simulink model "system_discrete"  (R2026b)
settings: Solver=VariableStepAuto  StopTime=50.0
values from neighbouring files (symbols this model uses):
  A_d = sys_d.A    [controller_observer_design.m]    (also in setup.m)
  B_d = sys_d.B    [controller_observer_design.m]    (also in setup.m)
  C_d = sys_d.C    [controller_observer_design.m]    (also in setup.m)
  K_discrete = dlqr(A_d,B_d,Q*Ts,R*Ts)    [controller_observer_design.m]    (also in setup.m)
  omega2u = [k, k, k, k; L*k, 0, -L*k, 0; 0, L*k, 0, -L*k; b, -b, b, -b]    [controller_observer_design.m]    (also in notes.m; setup.m)
  parameters =     [parameters.mat]
  Ts = 0.01    [controller_observer_design.m]    (also in setup.m)
  u2omega = (1/(4*b*L*k)) * [b*L, 2*b, 0, L*k; b*L, 0, 2*b, -L*k; b*L, -2*b, 0, L*k; b*L, 0, -2*b, -L*k]    [controller_observer_design.m]    (also in notes.m; setup.m)
undefined symbols (not defined in the file or in its folder): L_discrete
settings Model: Creator=elton  LastModifiedBy=elton

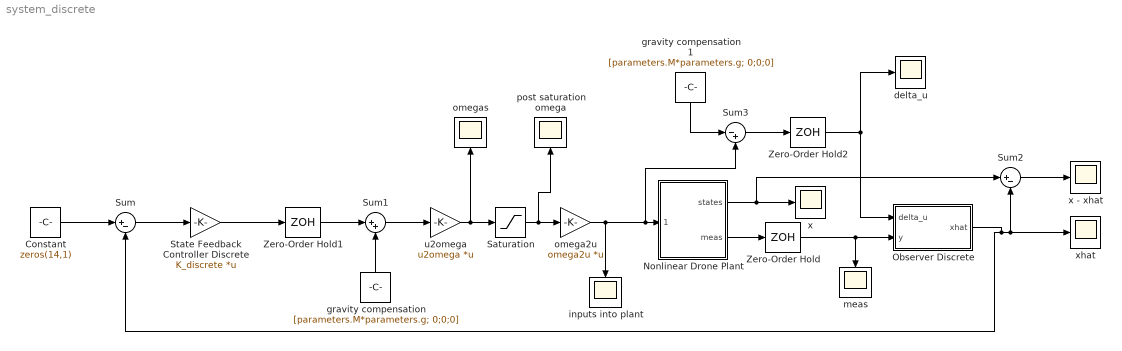
== system system_discrete ==
  Constant : Constant  Value=zeros(14,1)
  Nonlinear Drone Plant : Subsystem
  Observer Discrete : Subsystem
  Saturation : Saturate  UpperLimit=250000  LowerLimit=-250000
  State Feedback Controller Discrete : Gain  Gain=K_discrete  Multiplication=Matrix(K*u)
  Sum : Sum  Inputs=|+-
  Sum1 : Sum  Inputs=|++
  Sum2 : Sum  Inputs=|+-
  Sum3 : Sum  Inputs=|-+
  Zero-Order Hold : ZeroOrderHold  SampleTime=Ts
  Zero-Order Hold1 : ZeroOrderHold  SampleTime=Ts
  Zero-Order Hold2 : ZeroOrderHold  SampleTime=Ts
  delta_u : Scope
      settings: ActiveDisplayYMinimum=-0.1401923631580794  ActiveDisplayYMaximum=0.1652403175832419
  gravity compensation : Constant  Value=[parameters.M*parameters.g; 0;0;0]
  gravity compensation1 : Constant  Value=[parameters.M*parameters.g; 0;0;0]
  inputs into plant : Scope
      settings: ActiveDisplayYMinimum=-2.3883084159431922  ActiveDisplayYMaximum=20.39828479264926  DataLoggingVariableName=ScopeData7
  meas : Scope
      settings: ActiveDisplayYMinimum=-955.77756320006051  ActiveDisplayYMaximum=3490.5526217286788
  omega2u : Gain  Gain=omega2u  Multiplication=Matrix(K*u)
  omegas : Scope
      settings: ActiveDisplayYMinimum=134655.3751089205  ActiveDisplayYMaximum=149544.1079274721  DataLoggingVariableName=ScopeData8
  post saturation omega : Scope
      settings: ActiveDisplayYMinimum=131190.65308987262  ActiveDisplayYMaximum=153058.63070765982  DataLoggingVariableName=ScopeData9
  u2omega : Gain  Gain=u2omega  Multiplication=Matrix(K*u)
  x : Scope
      settings: ActiveDisplayYMinimum=-3.9919495753559691  ActiveDisplayYMaximum=4.13956426955115  DataLoggingVariableName=ScopeData6
  x - xhat : Scope
      settings: ActiveDisplayYMinimum=-0.067708761293840292  ActiveDisplayYMaximum=0.11746078567035534  DataLoggingVariableName=ScopeData2
  xhat : Scope
      settings: ActiveDisplayYMinimum=-0.014697140701710146  ActiveDisplayYMaximum=0.014411144567585507  DataLoggingVariableName=ScopeData3
  wires:
  Sum3/1 -> Zero-Order Hold2/1
  Sum1/1 -> u2omega/1
  State Feedback Controller Discrete/1 -> Zero-Order Hold1/1
  u2omega/1 -> Saturation/1, omegas/1
  omega2u/1 -> Sum3/2, Nonlinear Drone Plant/1(inputs), inputs into plant/1
  Observer Discrete/1(xhat) -> xhat/1, Sum2/2, Sum/2
  Nonlinear Drone Plant/1(states) -> x/1, Sum2/1
  Zero-Order Hold2/1 -> delta_u/1, Observer Discrete/1(delta_u)
  gravity compensation/1 -> Sum1/2
  Saturation/1 -> post saturation omega/1, omega2u/1
  gravity compensation1/1 -> Sum3/1
  Sum/1 -> State Feedback Controller Discrete/1
  Zero-Order Hold/1 -> meas/1, Observer Discrete/2(y)
  Sum2/1 -> x - xhat/1
  Zero-Order Hold1/1 -> Sum1/1
  Nonlinear Drone Plant/2(meas) -> Zero-Order Hold/1
  Constant/1 -> Sum/1

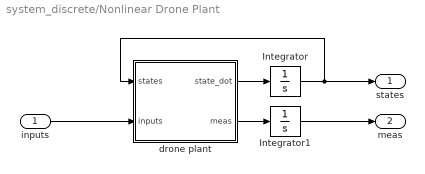
== system system_discrete/Nonlinear Drone Plant ==
  inputs : Inport
  Integrator : Integrator  InitialCondition=[zeros(12,1);0.049;0]
  Integrator1 : Integrator  InitialCondition=zeros(6,1)
  drone plant : MATLAB Function  TreatAsAtomicUnit=on
  states : Outport
  meas : Outport  Port=2
  wires:
  drone plant/1(state_dot) -> Integrator/1
  Integrator/1 -> states/1, drone plant/1(states)
  inputs/1 -> drone plant/2(inputs)
  Integrator1/1 -> meas/1
  drone plant/2(meas) -> Integrator1/1

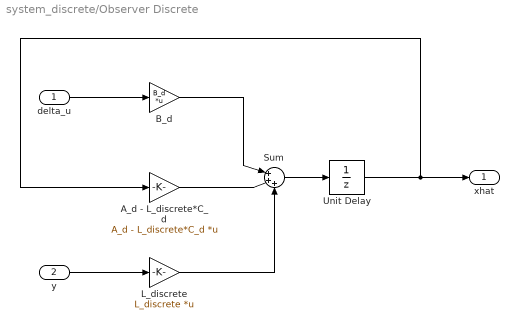
== system system_discrete/Observer Discrete ==
  delta_u : Inport
  y : Inport  Port=2
  A_d - L_discrete*C_d : Gain  Gain=A_d - L_discrete*C_d  Multiplication=Matrix(K*u)
  B_d : Gain  Gain=B_d  Multiplication=Matrix(K*u)
  L_discrete : Gain  Gain=L_discrete  Multiplication=Matrix(K*u)
  Sum : Sum  Inputs=|+++
  Unit Delay : UnitDelay  InitialCondition=zeros(14,1)  SampleTime=-1
  xhat : Outport
  wires:
  y/1 -> L_discrete/1
  B_d/1 -> Sum/1
  L_discrete/1 -> Sum/3
  A_d - L_discrete*C_d/1 -> Sum/2
  Sum/1 -> Unit Delay/1
  Unit Delay/1 -> A_d - L_discrete*C_d/1, xhat/1
  delta_u/1 -> B_d/1

== matlab function system_discrete/Nonlinear Drone Plant/drone plant ==
  data: states input size=14; inputs input size=4; state_dot output size=14; parameters parameter; meas output
%% non-linear state space
function [state_dot, meas]  = nonlin_state_space(states, inputs, parameters)
m     = parameters.m;
m_p    = parameters.m_p;
M     = m + m_p;
g     = parameters.g;
l     = parameters.l;
k_D    = parameters.k_D;
I_xx  = parameters.I_xx;
I_yy  = parameters.I_yy;
I_zz  = parameters.I_zz;

xi = states(1:3);
xi_dot = states(4:6);
eta = states(7:9);
nu = states(10:12);
alpha = states(13);
alpha_dot = states(14);

u_T = inputs(1);
tau = inputs(2:4);

x_dot = xi_dot(1);
y_dot = xi_dot(2);
z_dot = xi_dot(3);

% kinematics
phi = eta(1);
theta = eta(2);
psi = eta(3);
W_inv = [1,  sin(phi)*tan(theta), cos(phi)*tan(theta);
    0,  cos(phi),            -sin(phi);
    0,  sin(phi)/cos(theta), cos(phi)/cos(theta)];

eta_dot = W_inv*nu;

%rotational dynamics
p_dot = (tau(1)/I_xx) + ((I_yy-I_zz)/I_xx)*nu(2)*nu(3);
q_dot = (tau(2)/I_yy) + ((I_zz-I_xx)/I_yy)*nu(1)*nu(3);
r_dot = (tau(3)/I_zz) + ((I_xx-I_yy)/I_zz)*nu(1)*nu(2);
nu_dot = [p_dot; q_dot; r_dot];

%translational dynamics
c_alpha = cos(alpha);
s_alpha = sin(alpha);
c_phi = cos(phi); s_phi = sin(phi);
c_theta = cos(theta); s_theta = sin(theta);
c_psi = cos(psi); s_psi = sin(psi);

Fx = (c_psi*s_theta*c_phi + s_psi*s_phi) * u_T;
Fy = (s_psi*s_theta*c_phi - c_psi*s_phi) * u_T;
Fz = c_theta*c_phi * u_T;

x_dotdot = (1/(m*M)) * ( (m + m_p*c_alpha^2)*(Fx - k_D*x_dot) - m_p*s_alpha*c_alpha*(Fz - k_D*z_dot) + m*m_p*l*alpha_dot^2*s_alpha );
y_dotdot = (Fy - k_D*y_dot) / m;
z_dotdot = (1/(m*M)) * ( (m + m_p*s_alpha^2)*(Fz - k_D*z_dot) - m_p*s_alpha*c_alpha*(Fx - k_D*x_dot) + m*m_p*l*alpha_dot^2*c_alpha ) - g;
xi_dotdot = [x_dotdot; y_dotdot; z_dotdot];

% pendulum dynamics
%alpha_dotdot = (1 / (M * l)) * ( -Fx * c_alpha + Fz * s_alpha + k_D * x_dot * c_alpha - k_D * z_dot * s_alpha );
alpha_dotdot = (1/l)*(-x_dotdot*c_alpha - z_dotdot*s_alpha+g*s_alpha);

% assemble state_dot and meas
state_dot = [xi_dot; xi_dotdot; eta_dot; nu_dot; alpha_dot; alpha_dotdot];
meas = [xi_dot; eta_dot];
end
